simulink model "grasp_no_graphics"  (R2026a)
settings: Solver=daessc  StopTime=Run.timeout  MaxStep=0.001
undefined symbols (not defined in the file): C, km, Q, Run, U, X, Y, Z
libraries: sm_lib x80, nesl_utility x39, simulink x1
(part 3 of 3)

== matlab function grasp_no_graphics/Supervisor ==
  data: t input size=[1 1]; cmd output size=[9 1]; boxTarget input size=[9 1]; status input size=[20 1]; q input size=[7 1]; qf input size=[2 1]; qfd input size=[2 1]; gripCmd output size=[1 1]; sv output size=[14 1]; Run parameter; U parameter
function [cmd, gripCmd, sv] = supervisor(t, boxTarget, status, q, qf, qfd, Run, U)
% The 50 Hz grasp phases: grasp.supervisor.superviseGrasp.
persistent S
if isempty(S), S = grasp.supervisor.startingSupervisorState(); end
[cmd, gripCmd, sv, S] = grasp.supervisor.superviseGrasp(S, t, boxTarget, status, q, qf, qfd, Run.truth_grasp(:), U);

== matlab function grasp_no_graphics/Controller ==
  data: q input size=[7 1]; tau output size=[7 1]; qd input size=[7 1]; wRaw input size=[6 1]; cmd input size=[9 1]; gripCmd input size=[1 1]; qf input size=[2 1]; qfd input size=[2 1]; fFinger output size=[2 1]; status output size=[20 1]; C parameter; km parameter
function [tau, fFinger, status] = controller(q, qd, wRaw, cmd, gripCmd, qf, qfd, C, km)
% The 1 kHz arm and gripper controller: grasp.control.controlArm.
persistent S
if isempty(S), S = grasp.control.startingControlState(C); end
[tau, fFinger, status, S] = grasp.control.controlArm(S, q, qd, wRaw, cmd, gripCmd, qf, qfd, C, km);

== matlab function grasp_no_graphics/Box target ==
  data: t input size=[1 1]; boxTarget output size=[9 1]; phase input size=[1 1]; Run parameter; Q parameter
function boxTarget = boxTargetBlock(t, phase, Run, Q)
% Where the chosen box is: grasp.perception.knownBoxPose.
boxTarget = grasp.perception.knownBoxPose(t, phase, Run, Q);
